simulink model "TrajRunner"  (R2026a)
settings: Solver=ode4  StopTime=inf  FixedStep=1/500  EnableMultiTasking=on
undefined symbols (not defined in the file or in its folder): HIL, qc_get_step_size
libraries: quarc_library x14, simulink x1
settings Model: SimulationMode=external  ExtModeTrigDuration=10000  Creator=fvranes  LastModifiedBy=meow1
settings SolverCC: PositivePriorityOrder=on
settings RTWCC: SystemTargetFile=quarc_win64.tlc  TemplateMakefile=quarc_default_tmf  Toolchain=QUARC win64 | nmake (64-bit Windows)  BuildConfiguration=Faster Runs  Description=QUARC Win64 Target Using Toolchain
settings STFCustomTargetCC: SystemTargetFile=quarc_win64.tlc  MultiwordLength=2048.0  ConcurrentExecutionCompliant=on  UseToolchainInfoCompliant=on
settings GRTTargetCC: ExtMode=on  ExtModeMexFile=quarc_comm  ParMdlRefBuildCompliant=off  CompOptLevelCompliant=off  CombineOutputUpdateFcns=off  MatFileLogging=off  CPPClassGenCompliant=off  GRTInterface=on
settings ConfigComp: CovMetricSettings=dswe

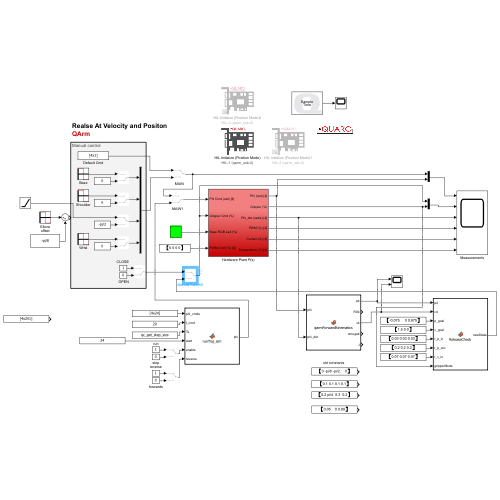
[thumbnail: Simulink's stored preview of the top-level diagram]
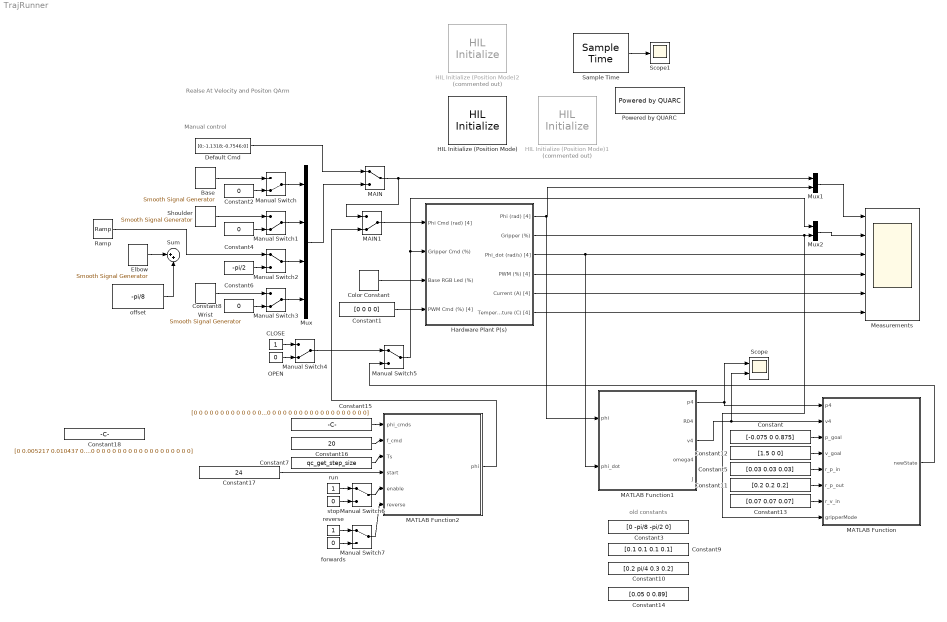
== system TrajRunner ==
  note: old constants
  note: Manual control
  note: Realse At Velocity and Positon
      | QArm
  " OPEN" : Constant  Value=0
  Base : quarc_library/Sources/Signals/Smooth Signal Generator  signal_type=Square  source=Internal (dialog parameters)  amplitude=pi/8  frequency=0.125  initial_phase=0  sample_time=qc_get_step_size  output_cos=off
      settings: SourceProductName=QUARC Targets
  "CLOSE " : Constant
  Color Constant : quarc_library/Sources/Signals/Color Constant  color=[0 1 0]
      settings: SourceProductName=QUARC Targets
  Constant : Constant  Value=[-0.075 0 0.875]
  Constant1 : Constant  Value=[0 0 0 0]
  Constant10 : Constant  Value=[0.2 pi/4 0.3 0.2]
  Constant11 : Constant  Value=[0.2 0.2 0.2]
  Constant12 : Constant  Value=[1.5 0 0]
  Constant13 : Constant  Value=[0.07 0.07 0.07]
  Constant14 : Constant  Value=[0.05 0 0.89]
  Constant15 : Constant  Value=[0 0 0 0 0 0 0 0 0 0 0 0 0 0 0 0 0 0 0 0 0 0 0 0;-1.13184 -1.13099 -1.12516 -1.10965 -1.08046 -1.03455 -0.97024 -0.88766 -0.78957 -0.68302 -0.5819 -0.50317 -0.45059 -0.41483 -0.38573 -0.36205 -0.34198 -0.32505 -0.31135 -0.30109 -0.29427 -0.29053 -0.2891 -0.28889;-0.75455 -0.75523 -0.75992 -0.77237 -0.79572 -0.83218 -0.88254 -0.94546 -1.01591 -1.082 -1.12002 -1.10135 -1.02304 -0.9073 -0.76354 -0.61795 -0.4826 -0.36555 -0.27168 -0.20284 -0.15808 -0.13389 -0.12468 -0.12334;0 0 0 0 0 0 0 0 0 0 0 0 0 0 0 0 0 0 0 0 0 0 0 0]
  Constant16 : Constant  Value=20
  Constant17 : Constant  Value=24
  Constant18 : Constant  Value=[0 0.005217 0.010437 0.015661 0.020889 0.02612 0.031251 0.036392 0.041544 0.046707 0.05188 0.056852 0.061842 0.066849 0.071872 0.076913 0.081653 0.086416 0.091202 0.096011 0.100842 0.105273 0.109732 0.114218 0.118731 0.123271 0.127314 0.131386 0.135488 0.139621 0.143784 0.147353 0.150952 0.154582 0.158244 0.161937 0.164943 0.167977 0.171041 0.174135 0.17726 0.179607 0.181979 0.184378 0.186802 0.189253 0.190843 0.192453 0.194081 0.195729 0.197396 0.19813 0.198873 0.199626 0.200388 0.20116 0.20094 0.200717 0.200491 0.200262 0.20003 0.198767 0.197486 0.19619 0.194876 0.193544 0.191166 0.188758 0.186319 0.183848 0.181344 0.177813 0.174239 0.170621 0.166958 0.16325 0.158573 0.153845 0.149064 0.144229 0.139341 0.13359 0.127786 0.121926 0.116011 0.110041 0.103364 0.096639 0.089865 0.083043 0.076173 0.068799 0.061392 0.05395 0.046476 0.038969 0.0312 0.023418 0.015623 0.007817 0 -0.007817 -0.015623 -0.023418 -0.0312 -0.038969 -0.046476 -0.05395 -0.061392 -0.068799 -0.076173 -0.083043 -0.089865 -0.096639 -0.103364 -0.110041 -0.116011 -0.121926 -0.127786 -0.13359 -0.139341 -0.144229 -0.149064 -0.153845 -0.158573 -0.16325 -0.166958 -0.170621 -0.174239 -0.177813 -0.181344 -0.183848 -0.186319 -0.188758 -0.191166 -0.193544 -0.194876 -0.19619 -0.197486 -0.198767 -0.20003 -0.200262 -0.200491 -0.200717 -0.20094 -0.20116 -0.200388 -0.199626 -0.198873 -0.19813 -0.197396 -0.195729 -0.194081 -0.192453 -0.190843 -0.189253 -0.186802 -0.184378 -0.181979 -0.179607 -0.17726 -0.174135 -0.171041 -0.167977 -0.164943 -0.161937 -0.158244 -0.154582 -0.150952 -0.147353 -0.143784 -0.139621 -0.135488 -0.131386 -0.127314 -0.123271 -0.118731 -0.114218 -0.109732 -0.105273 -0.100842 -0.096011 -0.091202 -0.086416 -0.081653 -0.076913 -0.071872 -0.066849 -0.061842 -0.056852 -0.05188 -0.046707 -0.041544 -0.036392 -0.031251 -0.02612 -0.020889 -0.015661 -0.010437 -0.005217 0;0.148643 0.148132 0.147657 0.147217 0.146812 0.146442 0.145059 0.143711 0.142397 0.141117 0.139871 0.137638 0.135438 0.133269 0.131132 0.129027 0.125979 0.122959 0.119968 0.117006 0.114072 0.110254 0.10646 0.10269 0.098945 0.095225 0.090693 0.086181 0.081688 0.077215 0.07276 0.067584 0.062421 0.057272 0.052135 0.047011 0.041269 0.035534 0.029805 0.024082 0.018365 0.012148 0.005931 -0.000287 -0.006506 -0.012726 -0.019314 -0.025909 -0.032511 -0.039121 -0.045739 -0.052579 -0.05943 -0.066295 -0.073173 -0.080064 -0.087018 -0.093987 -0.100972 -0.107973 -0.114991 -0.1219 -0.128824 -0.135764 -0.142721 -0.149694 -0.156376 -0.163069 -0.169775 -0.176493 -0.183224 -0.189474 -0.195727 -0.201985 -0.208246 -0.214512 -0.220106 -0.225693 -0.231271 -0.236841 -0.242402 -0.247109 -0.251795 -0.256457 -0.261095 -0.265709 -0.269308 -0.272869 -0.276392 -0.279875 -0.283318 -0.285617 -0.287865 -0.290062 -0.292207 -0.2943 -0.295164 -0.295969 -0.296716 -0.297404 -0.298033 -0.297404 -0.296716 -0.295969 -0.295164 -0.2943 -0.292207 -0.290062 -0.287865 -0.285617 -0.283318 -0.279875 -0.276392 -0.272869 -0.269308 -0.265709 -0.261095 -0.256457 -0.251795 -0.247109 -0.242402 -0.236841 -0.231271 -0.225693 -0.220106 -0.214512 -0.208246 -0.201985 -0.195727 -0.189474 -0.183224 -0.176493 -0.169775 -0.163069 -0.156376 -0.149694 -0.142721 -0.135764 -0.128824 -0.1219 -0.114991 -0.107973 -0.100972 -0.093987 -0.087018 -0.080064 -0.073173 -0.066295 -0.05943 -0.052579 -0.045739 -0.039121 -0.032511 -0.025909 -0.019314 -0.012726 -0.006506 -0.000287 0.005931 0.012148 0.018365 0.024082 0.029805 0.035534 0.041269 0.047011 0.052135 0.057272 0.062421 0.067584 0.07276 0.077215 0.081688 0.086181 0.090693 0.095225 0.098945 0.10269 0.10646 0.110254 0.114072 0.117006 0.119968 0.122959 0.125979 0.129027 0.131132 0.133269 0.135438 0.137638 0.139871 0.141117 0.142397 0.143711 0.145059 0.146442 0.146812 0.147217 0.147657 0.148132 0.148643;0.179029 0.179675 0.180278 0.180835 0.181348 0.181817 0.183565 0.185269 0.186928 0.188543 0.190113 0.192924 0.19569 0.198411 0.201089 0.203722 0.207529 0.211293 0.215013 0.218689 0.222321 0.227039 0.231713 0.236345 0.240933 ...(+1958 chars)]
  Constant2 : Constant  Value=0
  Constant3 : Constant  Value=[0 -pi/8 -pi/2 0]
  Constant4 : Constant  Value=0
  Constant5 : Constant  Value=[0.03 0.03 0.03]
  Constant6 : Constant  Value=-pi/2
  Constant7 : Constant  Value=qc_get_step_size
  Constant8 : Constant  Value=0
  Constant9 : Constant  Value=[0.1 0.1 0.1 0.1]
  Default Cmd : Constant  Value=[0;-1.1318;-0.7546;0]
  Elbow : quarc_library/Sources/Signals/Smooth Signal Generator  signal_type=Square  source=Internal (dialog parameters)  amplitude=pi/4  frequency=0.25  initial_phase=pi  sample_time=qc_get_step_size  output_cos=off
      settings: SourceProductName=QUARC Targets
  HIL Initialize (Position Mode) : quarc_library/Data Acquisition/Generic/Configuration/HIL Initialize  object_name=HIL-1  board_type=qarm_usb  board_number=0  board_options=j0_mode=0;j1_mode=0;j2_mode=0;j3_mode=0;gripper_mode=0;j0_profile_config=1;j0_profile_velocity=0.05;j0_profile_acceleration=0.01;j1_profile_config=1;j1_profile_velocity=0.05;j1_profile_acceleration=0.01;j2_profile_config=1;j2_profile_velocity=0.05;j2_profile_acceleration=0.01;j3_profile_config=1;j3_profile_velocity=0.05;j3_profile_acceleration=0.01;  exclusive=off  active=on  hardware_clocks=[0]  clock_modes=[]  initial_clock_frequencies=[]  set_clock_params_at_start=off  set_clock_params_at_switch_in=off  set_clock_frequencies_at_start=off  set_clock_frequencies_at_switch_in=off  analog_input_channels=[5:9]  analog_input_configurations=[]  analog_input_maximums=[]  analog_input_minimums=[]  set_analog_input_params_at_start=off  set_analog_input_params_at_switch_in=off  analog_output_channels=[]  analog_output_maximums=inf  analog_output_minimums=-inf  initial_analog_outputs=[0]  final_analog_outputs=[0]  watchdog_analog_outputs=[]  set_analog_output_params_at_start=off  set_analog_output_params_at_switch_in=off  set_analog_outputs_at_start=off  set_analog_outputs_at_switch_in=off  set_analog_outputs_at_terminate=off  set_analog_outputs_at_switch_out=off  set_analog_outputs_on_watchdog=off  digital_input_channels=[]  digital_output_channels=[]  digital_output_configuration=[]  initial_digital_outputs=[0]  final_digital_outputs=[0]  watchdog_digital_outputs=[0]  set_digital_output_params_at_start=off  set_digital_output_params_at_switch_in=off  set_digital_outputs_at_start=off  set_digital_outputs_at_switch_in=off  set_digital_outputs_at_terminate=off  set_digital_outputs_at_switch_out=off  set_digital_outputs_on_watchdog=off  encoder_channels=[]  quadrature=[]  encoder_filter_frequency=[]  initial_encoder_counts=[]  set_encoder_params_at_start=off  set_encoder_params_at_switch_in=off  set_encoder_counts_at_start=off  set_encoder_counts_at_switch_in=off  pwm_channels=[]  pwm_modes=[]  pwm_frequency=[]  pwm_configuration=[]  pwm_alignment=[]  pwm_polarity=[]  pwm_leading_deadband=[]  pwm_trailing_deadband=[]  initial_pwm_outputs=[]  final_pwm_outputs=[]  watchdog_pwm_outputs=[]  set_pwm_params_at_start=off  set_pwm_params_at_switch_in=off  set_pwm_outputs_at_start=off  set_pwm_outputs_at_switch_in=off  set_pwm_outputs_at_terminate=off  set_pwm_outputs_at_switch_out=off  set_pwm_outputs_on_watchdog=off  other_output_channels=[11005:11008 1000:1004 11000:11003]  initial_other_outputs=[zeros(1,9), ones(1,3)]  final_other_outputs=[1 0 0 0]  watchdog_other_outputs=zeros(1,12)  set_other_outputs_at_start=off  set_other_outputs_at_switch_in=off  set_other_outputs_at_terminate=on  set_other_outputs_at_switch_out=off  set_other_outputs_on_watchdog=off
  HIL Initialize (Position Mode)1 : quarc_library/Data Acquisition/Generic/Configuration/HIL Initialize  Commented=on  object_name=HIL-2  board_type=qarm_usb  board_number=0  board_options=j0_mode=0;j1_mode=0;j2_mode=0;j3_mode=0;gripper_mode=0;j0_profile_config=0;j0_profile_velocity=1.6;j0_profile_acceleration=1.0472;j1_profile_config=0;j1_profile_velocity=1.6;j1_profile_acceleration=1.0472;j2_profile_config=0;j2_profile_velocity=1.6;j2_profile_acceleration=1.0472;j3_profile_config=0;j3_profile_velocity=1.6;j3_profile_acceleration=1.0472;  exclusive=off  active=on  hardware_clocks=[0]  clock_modes=[]  initial_clock_frequencies=[]  set_clock_params_at_start=off  set_clock_params_at_switch_in=off  set_clock_frequencies_at_start=off  set_clock_frequencies_at_switch_in=off  analog_input_channels=[5:9]  analog_input_configurations=[]  analog_input_maximums=[]  analog_input_minimums=[]  set_analog_input_params_at_start=off  set_analog_input_params_at_switch_in=off  analog_output_channels=[]  analog_output_maximums=inf  analog_output_minimums=-inf  initial_analog_outputs=[0]  final_analog_outputs=[0]  watchdog_analog_outputs=[]  set_analog_output_params_at_start=off  set_analog_output_params_at_switch_in=off  set_analog_outputs_at_start=off  set_analog_outputs_at_switch_in=off  set_analog_outputs_at_terminate=off  set_analog_outputs_at_switch_out=off  set_analog_outputs_on_watchdog=off  digital_input_channels=[]  digital_output_channels=[]  digital_output_configuration=[]  initial_digital_outputs=[0]  final_digital_outputs=[0]  watchdog_digital_outputs=[0]  set_digital_output_params_at_start=off  set_digital_output_params_at_switch_in=off  set_digital_outputs_at_start=off  set_digital_outputs_at_switch_in=off  set_digital_outputs_at_terminate=off  set_digital_outputs_at_switch_out=off  set_digital_outputs_on_watchdog=off  encoder_channels=[]  quadrature=[]  encoder_filter_frequency=[]  initial_encoder_counts=[]  set_encoder_params_at_start=off  set_encoder_params_at_switch_in=off  set_encoder_counts_at_start=off  set_encoder_counts_at_switch_in=off  pwm_channels=[]  pwm_modes=[]  pwm_frequency=[]  pwm_configuration=[]  pwm_alignment=[]  pwm_polarity=[]  pwm_leading_deadband=[]  pwm_trailing_deadband=[]  initial_pwm_outputs=[]  final_pwm_outputs=[]  watchdog_pwm_outputs=[]  set_pwm_params_at_start=off  set_pwm_params_at_switch_in=off  set_pwm_outputs_at_start=off  set_pwm_outputs_at_switch_in=off  set_pwm_outputs_at_terminate=off  set_pwm_outputs_at_switch_out=off  set_pwm_outputs_on_watchdog=off  other_output_channels=[11005:11008 1000:1004 11000:11003]  initial_other_outputs=[zeros(1,9), ones(1,3)]  final_other_outputs=[1 0 0 0]  watchdog_other_outputs=zeros(1,12)  set_other_outputs_at_start=off  set_other_outputs_at_switch_in=off  set_other_outputs_at_terminate=on  set_other_outputs_at_switch_out=off  set_other_outputs_on_watchdog=off
  HIL Initialize (Position Mode)2 : quarc_library/Data Acquisition/Generic/Configuration/HIL Initialize  Commented=on  object_name=HIL-2  board_type=qarm_usb  board_number=0  board_options=j0_mode=0;j1_mode=0;j2_mode=0;j3_mode=0;gripper_mode=0;j0_profile_config=1;j0_profile_velocity=0.05;j0_profile_acceleration=0.01;j1_profile_config=1;j1_profile_velocity=0.05;j1_profile_acceleration=0.01;j2_profile_config=1;j2_profile_velocity=0.05;j2_profile_acceleration=0.01;j3_profile_config=1;j3_profile_velocity=0.05;j3_profile_acceleration=0.01;  exclusive=off  active=on  hardware_clocks=[0]  clock_modes=[]  initial_clock_frequencies=[]  set_clock_params_at_start=off  set_clock_params_at_switch_in=off  set_clock_frequencies_at_start=off  set_clock_frequencies_at_switch_in=off  analog_input_channels=[5:9]  analog_input_configurations=[]  analog_input_maximums=[]  analog_input_minimums=[]  set_analog_input_params_at_start=off  set_analog_input_params_at_switch_in=off  analog_output_channels=[]  analog_output_maximums=inf  analog_output_minimums=-inf  initial_analog_outputs=[0]  final_analog_outputs=[0]  watchdog_analog_outputs=[]  set_analog_output_params_at_start=off  set_analog_output_params_at_switch_in=off  set_analog_outputs_at_start=off  set_analog_outputs_at_switch_in=off  set_analog_outputs_at_terminate=off  set_analog_outputs_at_switch_out=off  set_analog_outputs_on_watchdog=off  digital_input_channels=[]  digital_output_channels=[]  digital_output_configuration=[]  initial_digital_outputs=[0]  final_digital_outputs=[0]  watchdog_digital_outputs=[0]  set_digital_output_params_at_start=off  set_digital_output_params_at_switch_in=off  set_digital_outputs_at_start=off  set_digital_outputs_at_switch_in=off  set_digital_outputs_at_terminate=off  set_digital_outputs_at_switch_out=off  set_digital_outputs_on_watchdog=off  encoder_channels=[]  quadrature=[]  encoder_filter_frequency=[]  initial_encoder_counts=[]  set_encoder_params_at_start=off  set_encoder_params_at_switch_in=off  set_encoder_counts_at_start=off  set_encoder_counts_at_switch_in=off  pwm_channels=[]  pwm_modes=[]  pwm_frequency=[]  pwm_configuration=[]  pwm_alignment=[]  pwm_polarity=[]  pwm_leading_deadband=[]  pwm_trailing_deadband=[]  initial_pwm_outputs=[]  final_pwm_outputs=[]  watchdog_pwm_outputs=[]  set_pwm_params_at_start=off  set_pwm_params_at_switch_in=off  set_pwm_outputs_at_start=off  set_pwm_outputs_at_switch_in=off  set_pwm_outputs_at_terminate=off  set_pwm_outputs_at_switch_out=off  set_pwm_outputs_on_watchdog=off  other_output_channels=[11005:11008 1000:1004 11000:11003]  initial_other_outputs=[zeros(1,9), ones(1,3)]  final_other_outputs=[1 0 0 0]  watchdog_other_outputs=zeros(1,12)  set_other_outputs_at_start=off  set_other_outputs_at_switch_in=off  set_other_outputs_at_terminate=on  set_other_outputs_at_switch_out=off  set_other_outputs_on_watchdog=off
  Hardware Plant P(s) : Subsystem
  MAIN : ManualSwitch
  MAIN1 : ManualSwitch  CurrentSetting=0
  MATLAB Function : MATLAB Function  TreatAsAtomicUnit=on
  MATLAB Function1 : MATLAB Function  TreatAsAtomicUnit=on
  MATLAB Function2 : MATLAB Function  TreatAsAtomicUnit=on
  Manual Switch{,1,3..4} (4 alike) : ManualSwitch  CurrentSetting=0
  Manual Switch{2,5..7} (4 alike) : ManualSwitch
  Measurements : Scope  NumInputPorts=6
      settings: TimeSpan=20  Title=Phi (angular position)  ActiveDisplayYMinimum=-3.4987236992312876  ActiveDisplayYMaximum=31.465497962286065  YLabel=degrees
  Mux : Mux
  Mux1 : Mux  Inputs=2
  Mux2 : Mux  Inputs=2
  Powered by QUARC : quarc_library/Logos/Powered by QUARC
  Ramp : simulink/Sources/Ramp  slope=pi/12  start=0  InitialOutput=0
  Sample Time : quarc_library/Sources/Time/Sample Time  Priority=-99  sample_time=qc_get_step_size
  Scope : Scope  NumInputPorts=2
      settings: ActiveDisplayYMinimum=-1.2318993556047713  ActiveDisplayYMaximum=1.6986768479440566  DataLoggingVariableName=ScopeData2
  Scope1 : Scope
      settings: ActiveDisplayYMinimum=0.00125  ActiveDisplayYMaximum=0.00274
  Shoulder : quarc_library/Sources/Signals/Smooth Signal Generator  signal_type=Square  source=Internal (dialog parameters)  amplitude=pi/3  frequency=0.25  initial_phase=0  sample_time=qc_get_step_size  output_cos=off
      settings: SourceProductName=QUARC Targets
  Sum : Sum  Inputs=|++
  Wrist : quarc_library/Sources/Signals/Smooth Signal Generator  signal_type=Square  source=Internal (dialog parameters)  amplitude=pi/8  frequency=0.125  initial_phase=0  sample_time=qc_get_step_size  output_cos=off
      settings: SourceProductName=QUARC Targets
  forwards : Constant  Value=0
  offset : Constant  Value=-pi/8
  reverse : Constant
  run : Constant
  stop : Constant  Value=0
  wires:
  Color Constant/1 -> Hardware Plant P(s)/3(Base RGB Led (%))
  Constant2/1 -> Manual Switch/2
  Constant4/1 -> Manual Switch1/2
  Constant6/1 -> Manual Switch2/2
  Constant8/1 -> Manual Switch3/2
  Wrist/1 -> Manual Switch3/1
  Manual Switch2/1 -> Mux/3
  Manual Switch3/1 -> Mux/4
  Manual Switch1/1 -> Mux/2
  Manual Switch/1 -> Mux/1
  Mux/1 -> MAIN/2
  Default Cmd/1 -> MAIN/1
  MAIN/1 -> Mux1/1, MAIN1/1
  "CLOSE "/1 -> Manual Switch4/1
  Base/1 -> Manual Switch/1
  Shoulder/1 -> Manual Switch1/1
  Elbow/1 -> Sum/1
  Constant1/1 -> Hardware Plant P(s)/4(PWM Cmd (%) [4])
  Sample Time/1 -> Scope1/1
  " OPEN"/1 -> Manual Switch4/2
  Hardware Plant P(s)/2(Gripper (%)) -> Mux2/2, MATLAB Function/8(gripperMode)
  Constant/1 -> MATLAB Function/3(p_goal)
  Constant5/1 -> MATLAB Function/5(r_p_in)
  Hardware Plant P(s)/1(Phi (rad) [4]) -> Mux1/2, MATLAB Function1/1(phi)
  Hardware Plant P(s)/3(Phi_dot (rad/s) [4]) -> MATLAB Function1/2(phi_dot), Measurements/3
  Mux2/1 -> Measurements/2
  Mux1/1 -> Measurements/1
  Hardware Plant P(s)/4(PWM (%) [4]) -> Measurements/4
  Hardware Plant P(s)/5(Current (A) [4]) -> Measurements/5
  Hardware Plant P(s)/6(Temperature (C) [4]) -> Measurements/6
  Manual Switch4/1 -> Manual Switch5/1
  MATLAB Function/1(newState) -> Manual Switch5/2
  Manual Switch5/1 -> Mux2/1, Hardware Plant P(s)/2(Gripper Cmd (%))
  offset/1 -> Sum/2
  MATLAB Function1/1(p4) -> Scope/1, MATLAB Function/1(p4)
  MATLAB Function1/3(v4) -> Scope/2, MATLAB Function/2(v4)
  Constant11/1 -> MATLAB Function/6(r_p_out)
  Constant12/1 -> MATLAB Function/4(v_goal)
  Constant13/1 -> MATLAB Function/7(r_v_in)
  Constant7/1 -> MATLAB Function2/3(Ts)
  Constant15/1 -> MATLAB Function2/1(phi_cmds)
  MAIN1/1 -> Hardware Plant P(s)/1(Phi Cmd (rad) [4])
  Ramp/1 -> Manual Switch2/1
  Constant16/1 -> MATLAB Function2/2(f_cmd)
  MATLAB Function2/1(phi) -> MAIN1/2
  run/1 -> Manual Switch6/1
  stop/1 -> Manual Switch6/2
  Manual Switch6/1 -> MATLAB Function2/5(enable)
  forwards/1 -> Manual Switch7/2
  reverse/1 -> Manual Switch7/1
  Manual Switch7/1 -> MATLAB Function2/6(reverse)
  Constant17/1 -> MATLAB Function2/4(start)

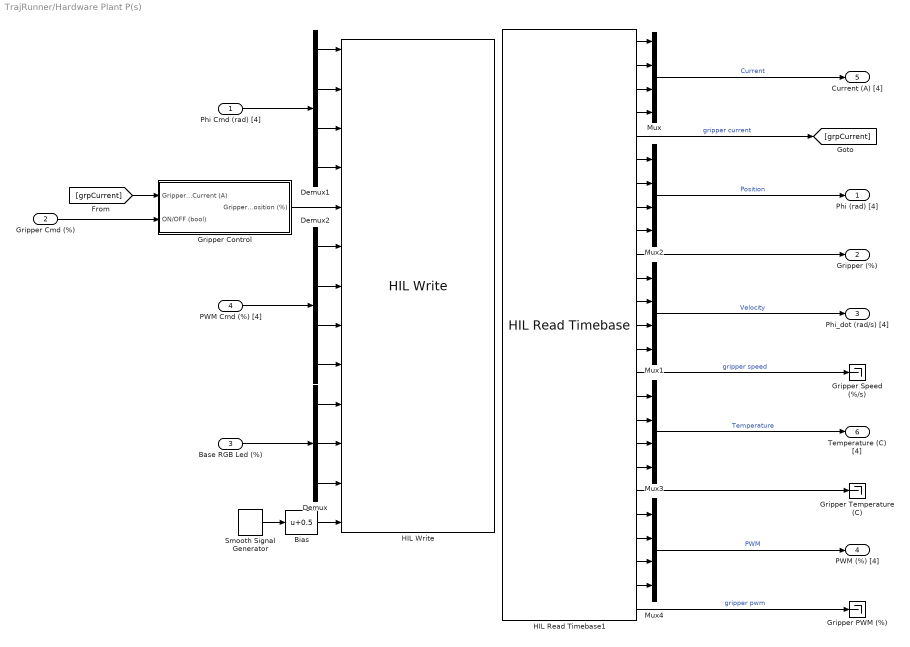
== system TrajRunner/Hardware Plant P(s) ==
  Phi Cmd (rad) [4] : Inport
  Gripper Cmd (%) : Inport  Port=2
  Base RGB Led (%) : Inport  Port=3
  PWM Cmd (%) [4] : Inport  Port=4
  Bias : Bias  Bias=0.5  SaturateOnIntegerOverflow=off
  Demux : Demux  Outputs=3
  Demux1 : Demux
  Demux2 : Demux
  Gripper Control : Subsystem
  Gripper PWM (%) : Terminator
  Gripper Speed (%/s) : Terminator
  Gripper Temperature (C) : Terminator
  HIL Read Timebase1 : quarc_library/Data Acquisition/Generic/Timebases/HIL Read Timebase  object_name=HIL-1  clock=0  analog_channels=[5:9]  encoder_channels=[]  digital_channels=[]  other_channels=[1000:1004 3000:3004 10000:10004 11000:11004]  active=on  vector_output=off  port_labels=channel numbers  data_type_mode=Inherit via back propagation  encoder_data_type=double  digital_data_type=boolean  overflow_mode=Error on overflow  samples_in_buffer=max(ceil(1/qc_get_step_size), 1)
  HIL Write : quarc_library/Data Acquisition/Generic/Immediate I//O/HIL Write  object_name=HIL-1  analog_channels=[]  pwm_channels=[]  digital_channels=[]  other_channels=[1000:1004 11000:11003 11005:11008]  sample_time=-1  active=on  vector_input=off  port_labels=channel numbers
  Mux{,1..4} (5 alike) : Mux
  Smooth Signal Generator : quarc_library/Sources/Signals/Smooth Signal Generator  signal_type=Sine  source=Internal (dialog parameters)  amplitude=0.5  frequency=0.5  initial_phase=0  sample_time=qc_get_step_size  output_cos=off
      settings: SourceProductName=QUARC Targets
  Phi (rad) [4] : Outport  VectorParamsAs1DForOutWhenUnconnected=off
  Gripper (%) : Outport  Port=2  VectorParamsAs1DForOutWhenUnconnected=off
  Phi_dot (rad/s) [4] : Outport  Port=3  VectorParamsAs1DForOutWhenUnconnected=off
  PWM (%) [4] : Outport  Port=4  VectorParamsAs1DForOutWhenUnconnected=off
  Current (A) [4] : Outport  Port=5  VectorParamsAs1DForOutWhenUnconnected=off
  Temperature (C) [4] : Outport  Port=6  VectorParamsAs1DForOutWhenUnconnected=off
  wires:
  Gripper Cmd (%)/1 -> Gripper Control/2(ON/OFF (bool))
  HIL Read Timebase1/10 -> Gripper (%)/1
  Mux4/1 -> PWM (%) [4]/1  "PWM"
  HIL Read Timebase1/25 -> Gripper PWM (%)/1  "gripper pwm"
  HIL Read Timebase1/24 -> Mux4/4
  HIL Read Timebase1/23 -> Mux4/3
  HIL Read Timebase1/22 -> Mux4/2
  HIL Read Timebase1/21 -> Mux4/1
  Mux2/1 -> Phi (rad) [4]/1  "Position"
  Demux2/4 -> HIL Write/9
  Demux2/3 -> HIL Write/8
  Demux2/2 -> HIL Write/7
  Demux2/1 -> HIL Write/6
  PWM Cmd (%) [4]/1 -> Demux2/1
  Phi Cmd (rad) [4]/1 -> Demux1/1
  Demux1/4 -> HIL Write/4
  Demux1/3 -> HIL Write/3
  Demux1/2 -> HIL Write/2
  Demux1/1 -> HIL Write/1
  Base RGB Led (%)/1 -> Demux/1
  Mux3/1 -> Temperature (C) [4]/1  "Temperature"
  Mux1/1 -> Phi_dot (rad/s) [4]/1  "Velocity"
  Mux/1 -> Current (A) [4]/1  "Current"
  HIL Read Timebase1/20 -> Gripper Temperature (C)/1
  HIL Read Timebase1/1 -> Mux/1
  HIL Read Timebase1/2 -> Mux/2
  HIL Read Timebase1/13 -> Mux1/3
  Demux/2 -> HIL Write/11
  HIL Read Timebase1/19 -> Mux3/4
  Demux/1 -> HIL Write/10
  HIL Read Timebase1/11 -> Mux1/1
  HIL Read Timebase1/16 -> Mux3/1
  HIL Read Timebase1/17 -> Mux3/2
  HIL Read Timebase1/3 -> Mux/3
  Demux/3 -> HIL Write/12
  HIL Read Timebase1/15 -> Gripper Speed (%/s)/1  "gripper speed"
  HIL Read Timebase1/5 -> [grpCurrent]  "gripper current"
  HIL Read Timebase1/7 -> Mux2/2
  HIL Read Timebase1/4 -> Mux/4
  HIL Read Timebase1/12 -> Mux1/2
  HIL Read Timebase1/8 -> Mux2/3
  HIL Read Timebase1/18 -> Mux3/3
  HIL Read Timebase1/6 -> Mux2/1
  HIL Read Timebase1/9 -> Mux2/4
  HIL Read Timebase1/14 -> Mux1/4
  Smooth Signal Generator/1 -> Bias/1
  Bias/1 -> HIL Write/13
  Gripper Control/1(Gripper Position (%)) -> HIL Write/5
  [grpCurrent] -> Gripper Control/1(Gripper Current (A))

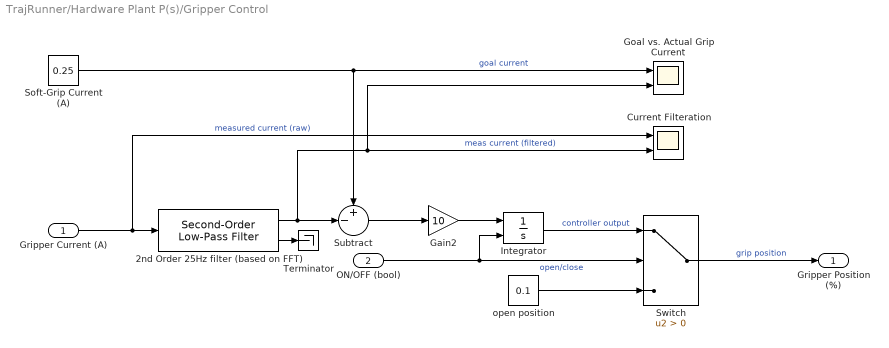
== system TrajRunner/Hardware Plant P(s)/Gripper Control ==
  Gripper Current (A) : Inport
  ON/OFF (bool) : Inport  Port=2
  2nd Order 25Hz filter (based on FFT) : quarc_library/Continuous/Second-Order Low-Pass Filter  params_source=Internal (dialog parameters)  input_width=25*2*pi  input_zeta=1  input_init=0
  Current Filteration : Scope  NumInputPorts=2
      settings: ActiveDisplayYMinimum=-0.01447  ActiveDisplayYMaximum=0.62651  DataLoggingVariableName=ScopeData5
  Gain2 : Gain  Gain=10
  Goal vs. Actual Grip Current : Scope  NumInputPorts=2
      settings: ActiveDisplayYMinimum=0.00229  ActiveDisplayYMaximum=0.27702  DataLoggingVariableName=ScopeData4
  Integrator : Integrator  ExternalReset=either  InitialCondition=0.1  LimitOutput=on  UpperSaturationLimit=0.9  LowerSaturationLimit=0.1
  Soft-Grip Current (A) : Constant  Value=0.25
  Subtract : Sum  Inputs=+-|
  Switch : Switch  Criteria=u2 > Threshold  SaturateOnIntegerOverflow=off  InputSameDT=off
  Terminator : Terminator
  open position : Constant  Value=0.1
  Gripper Position (%) : Outport  VectorParamsAs1DForOutWhenUnconnected=off
  wires:
  Gripper Current (A)/1 -> 2nd Order 25Hz filter (based on FFT)/1, Current Filteration/1  "measured current (raw)"
  ON/OFF (bool)/1 -> Switch/2, Integrator/2  "open/close"
  open position/1 -> Switch/3
  Switch/1 -> Gripper Position (%)/1  "grip position"
  Soft-Grip Current (A)/1 -> Subtract/1, Goal vs. Actual Grip Current/1  "goal current"
  2nd Order 25Hz filter (based on FFT)/1 -> Subtract/2, Current Filteration/2, Goal vs. Actual Grip Current/2  "meas current (filtered)"
  Subtract/1 -> Gain2/1
  Integrator/1 -> Switch/1  "controller output"
  Gain2/1 -> Integrator/1
  2nd Order 25Hz filter (based on FFT)/2 -> Terminator/1

== matlab function TrajRunner/MATLAB Function1 ==
  data: phi input; p4 output; R04 output; v4 output; omega4 output; J output; phi_dot input
function [p4, R04, v4, omega4, J] = qarmForwardKinematics(phi, phi_dot)
%QARMFORWARDKINEMATICS Compute the QArm end-effector pose and velocity.
%   phi is the 4-by-1 vector of physical QArm joint angles (rad).
%   phi_dot is the 4-by-1 vector of physical joint velocities (rad/s).
%   p4 is the end-effector position (m) in frame {0}, and R04 is its
%   orientation. v4 is the linear velocity of p4 (m/s), and omega4 is
%   the end-effector angular velocity (rad/s), both expressed in frame {0}.
%   J is the 6-by-4 geometric Jacobian: [v4; omega4] = J*phi_dot.
%   The original call [p4, R04] = qarmForwardKinematics(phi) still works.
%   If phi_dot is omitted, v4 and omega4 are returned as empty arrays.

validateattributes(phi, {'numeric'}, {'real', 'finite', 'vector', 'numel', 4}, ...
    mfilename, 'phi', 1);
phi = phi(:);
if nargin >= 2
    validateattributes(phi_dot, {'numeric'}, ...
        {'real', 'finite', 'vector', 'numel', 4}, mfilename, 'phi_dot', 2);
    phi_dot = phi_dot(:);
end

% Manipulator dimensions (m)
L1 = 0.1400;
L2 = 0.3500;
L3 = 0.0500;
L4 = 0.2500;
L5 = 0.1500;

% Equivalent geometric parameters
l1 = L1;
l2 = sqrt(L2^2 + L3^2);
l3 = L4 + L5;
beta = atan(L3/L2);

% Convert the physical joint coordinates phi to DH coordinates theta.
theta = phi;
theta(1) = phi(1);
theta(2) = phi(2) + beta - pi/2;
theta(3) = phi(3) - beta;
theta(4) = phi(4);

% Standard DH table:
% i       a_i       alpha_i       d_i       theta_i
% 1        0          -pi/2        l1        theta(1)
% 2        l2          0            0        theta(2)
% 3        0          -pi/2         0        theta(3)
% 4        0           0            l3       theta(4)
T01 = quanser_arm_DH(0,  -pi/2, l1, theta(1));
T12 = quanser_arm_DH(l2,  0,     0, theta(2));
T23 = quanser_arm_DH(0,  -pi/2,  0, theta(3));
T34 = quanser_arm_DH(0,   0,    l3, theta(4));

T02 = T01*T12;
T03 = T02*T23;
T04 = T03*T34;

p4 = T04(1:3, 4);
R04 = T04(1:3, 1:3);

% Joint i rotates about z_{i-1}. Express each axis and origin in frame {0}.
p0 = [0; 0; 0];
p1 = T01(1:3, 4);
p2 = T02(1:3, 4);
p3 = T03(1:3, 4);
z0 = [0; 0; 1];
z1 = T01(1:3, 3);
z2 = T02(1:3, 3);
z3 = T03(1:3, 3);

% Revolute-joint Jacobian columns: z_{i-1} cross (p4 - p_{i-1}).
% The DH angles differ from phi only by constant offsets, so
% theta_dot = phi_dot and no additional coordinate conversion is needed.
Jv = [cross(z0, p4-p0), cross(z1, p4-p1), ...
      cross(z2, p4-p2), cross(z3, p4-p3)];
Jw = [z0, z1, z2, z3];
J = [Jv; Jw];

if nargin >= 2
    v4 = Jv*phi_dot;
    omega4 = Jw*phi_dot;
else
    v4 = [];
    omega4 = [];
end
end

function T = quanser_arm_DH(a, alpha, d, theta)
%QUANSER_ARM_DH Standard DH homogeneous transform.
T_R_z = [cos(theta), -sin(theta), 0, 0;
         sin(theta),  cos(theta), 0, 0;
         0,           0,          1, 0;
         0,           0,          0, 1];

T_T_z = [1, 0, 0, 0;
         0, 1, 0, 0;
         0, 0, 1, d;
         0, 0, 0, 1];

T_T_x = [1, 0, 0, a;
         0, 1, 0, 0;
         0, 0, 1, 0;
         0, 0, 0, 1];

T_R_x = [1, 0,          0,           0;
         0, cos(alpha), -sin(alpha), 0;
         0, sin(alpha),  cos(alpha), 0;
         0, 0,           0,           1];

T = T_R_z*T_T_z*T_T_x*T_R_x;
end

== matlab function TrajRunner/MATLAB Function ==
  data: p4 input; v4 input; newState output; p_goal input; v_goal input; r_p_in input; r_p_out input; r_v_in input; gripperMode input
function newState  = ReleaseCheck(p4, v4, p_goal, v_goal, r_p_in, r_p_out, r_v_in, gripperMode)
%#codegen
% Determines the state of the gripper on the QArm based on the end-effector
% position and velocity output by qarmForwardKinematics. The object is
% released when the end effector reaches the goal position AND the goal
% velocity. Uses hysteresis to prevent chattering.
% Inputs:
%   p4          - 3x1 end-effector position in frame {0} (m)
%   v4          - 3x1 end-effector linear velocity in frame {0} (m/s)
%   p_goal      - 3x1 goal end-effector position in frame {0} (m)
%   v_goal      - 3x1 goal end-effector velocity in frame {0} (m/s)
%   r_p_in      - inner position tolerance (per axis, m); every axis must be
%                 inside this to release the gripper (1 -> 0)
%   r_p_out     - outer position tolerance (per axis, m); any axis leaving
%                 this closes the gripper again (0 -> 1)
%                 (r_p_out > r_p_in creates the hysteresis band)
%   r_v_in      - velocity tolerance (per axis, m/s); every axis of the
%                 velocity error must be inside this to release
%   gripperMode - current gripper state (0 or 1) 0 is open and 1 is closed
% Output:
%   newState    - updated gripper state (0 or 1)



    checkVel = [1;1;1];
%               - velocity check enable flag(s). Scalar: 1 checks velocity
%                 on all axes, 0 ignores velocity. 3x1: enables the check
%                 per axis, e.g. [1;0;0] only checks the x velocity

    % calculate Cartesian position and velocity error
    p_err = p_goal(:) - p4(:);
    v_err = v_goal(:) - v4(:);

    if (gripperMode > 0.5)
        gripperMode = 1;
    else
        gripperMode = 0;
    end
    % default: hold the current state
    newState = gripperMode;

    if gripperMode == 1
        % release only when EVERY axis is inside the inner band and the
        % end effector is moving at (nearly) the goal velocity. Axes with
        % the velocity check disabled always pass.
        velOk = (abs(v_err) <= r_v_in(:)) | ~logical(checkVel(:));
        inside = all(abs(p_err) <= r_p_in(:)) && all(velOk);
        if inside
            newState = 0;
        end

    else
        % close again when ANY axis leaves the outer band
        outside = any(abs(p_err) >= r_p_out(:));
        if outside
            newState = 1;
        end
    end

end

== matlab function TrajRunner/MATLAB Function2 ==
  data: phi_cmds input; phi output; f_cmd input; Ts input; start input; enable input; reverse input
function phi  = runTraj_sim(phi_cmds, f_cmd, Ts, start, enable, reverse)
phi = runTraj(phi_cmds, f_cmd, Ts, start, enable, reverse)
